simulink model "ACFT11_a_121_precoast_backup"  (R2026a)
settings: Solver=ode15s  StopTime=2200  FixedStep=0.01  MaxStep=0.05  MinStep=1e-4  AbsTol=1e-4
model workspace (MAT data in the model file):
  op11 : opcond.OperatingPoint (value not decoded)
  op_trim1 : opcond.OperatingReport (value not decoded)
  op_trim12 : opcond.OperatingReport (value not decoded)
  op_trim15 : opcond.OperatingReport (value not decoded)
  op_trim16 : opcond.OperatingReport (value not decoded)
  op_trim17 : opcond.OperatingReport (value not decoded)
  op_trim18 : opcond.OperatingReport (value not decoded)
  op_trim2 : opcond.OperatingReport (value not decoded)
  op_trim20 : opcond.OperatingReport (value not decoded)
  op_trim21 : opcond.OperatingReport (value not decoded)
  op_trim22 : opcond.OperatingReport (value not decoded)
  op_trim23 : opcond.OperatingReport (value not decoded)
  op_trim24 : opcond.OperatingReport (value not decoded)
  op_trim25 : opcond.OperatingReport (value not decoded)
  op_trim29 : opcond.OperatingReport (value not decoded)
  op_trim3 : opcond.OperatingReport (value not decoded)
  op_trim30 : opcond.OperatingReport (value not decoded)
  op_trim4 : opcond.OperatingReport (value not decoded)
  op_trim40 : opcond.OperatingReport (value not decoded)
  op_trim42 : opcond.OperatingReport (value not decoded)
  op_trim5 : opcond.OperatingReport (value not decoded)
  op_trim50 : opcond.OperatingReport (value not decoded)
  op_trim7 : opcond.OperatingReport (value not decoded)
  op_trim9 : opcond.OperatingReport (value not decoded)
values from neighbouring files (symbols this model uses):
  b = min(1, 2*(1-frac))    [export_kml.m]    (also in flight_hud.m = chaseBack; inertiatensor62.m = 9.05; setup_bfl_analysis.m = 9.05; setup_fcs_sim.m = 9.05)
  c = bar_colors{min(k,numel(bar_colors))}    [analyze_bfl.m]    (also in ecef_eom_fcn.m = w_eb_b(3); inertiatensor62.m = 15.55; optimize_indi_gains.m = 15.55; restore_normal_fcs.m = 15.55)
  CL_AlphaDot = 0    [inertiatensor62.m]    (also in setup_bfl_analysis.m; setup_fcs_sim.m; setup_takeoff_fcs.m)
  Cm_AlphaDot = 0    [inertiatensor62.m]    (also in setup_bfl_analysis.m; setup_fcs_sim.m; setup_takeoff_fcs.m)
  ecef_x0 = [ [0;0;0]; ECEF_v0; ECEF_q0; ECEF_w0 ]    [setup_ecef.m]    (also in setup_fcs_sim.m = build_ecef_x0(FCS_h_cmd, FCS_V_cmd, 2*pi/180))
  F = convhull(pts)    [Visualization_Takeoff2.m]    (also in attitude_ribbon.m = {[1 2 3],[1 4 2],[1 4 3],[4 5 1]})
  FCS_aerospike_thrust = 250000.0    (= 250000)    [fcs_params.m]
  FCS_alpha_max = 16.0    (= 16)    [fcs_params.m]
  FCS_bank_max = 35.0    (= 35)    [fcs_params.m]
  FCS_da_max = 20.0    (= 20)    [fcs_params.m]
  FCS_de_max = 25.0    (= 25)    [fcs_params.m]
  FCS_dr_max = 25.0    (= 25)    [fcs_params.m]
  FCS_dt = 0.01    [fcs_params.m]
  FCS_g = 9.80665    [fcs_params.m]
  FCS_Gmin_p = 0.02    [fcs_params.m]
  FCS_Gmin_q = 0.02    [fcs_params.m]
  FCS_Gmin_r = 0.01    [fcs_params.m]
  FCS_h_gnd = 2.24    [fcs_params.m]
  FCS_hdot_max = 30.0    (= 30)    [fcs_params.m]
  FCS_hdot_td = 0.3    [fcs_params.m]
  FCS_Kalpha = 3.0    (= 3)    [fcs_params.m]
  FCS_Kalpha_lim = 2.0    (= 2)    [fcs_params.m]
  FCS_Kbeta = 2.0    (= 2)    [fcs_params.m]
  FCS_Kflare = 1.0    (= 1)    [fcs_params.m]
  FCS_Kgamma = 1.5    [fcs_params.m]
  FCS_Kh = 0.10    (= 0.1)    [fcs_params.m]
  FCS_Knz = 20.0    (= 20)    [fcs_params.m]
  FCS_Kp = 6.0    (= 6)    [fcs_params.m]
  FCS_Kphi = 3.0    (= 3)    [fcs_params.m]
  FCS_Kq = 5.0    (= 5)    [fcs_params.m]
  FCS_Kr = 4.0    (= 4)    [fcs_params.m]
  FCS_Ktheta = 2.0    (= 2)    [fcs_params.m]
  FCS_link_timeout = 1.0    (= 1)    [fcs_params.m]
  FCS_MODE_AUTO = 0    [fcs_params.m]
  FCS_Nfilt = 20.0    (= 20)    [fcs_params.m]
  FCS_Nz_max = 3.0    (= 3)    [fcs_params.m]
  FCS_Nz_min = -1.0    (= -1)    [fcs_params.m]
  FCS_Nz_zoom_tgt = 2.0    (= 2)    [fcs_params.m]
  FCS_p_max = 40.0    (= 40)    [fcs_params.m]
  FCS_q_max = 15.0    (= 15)    [fcs_params.m]
  FCS_qbar_hi = 6000.0    (= 6000)    [fcs_params.m]
  FCS_qbar_lo = 1000.0    (= 1000)    [fcs_params.m]
  FCS_r_max = 15.0    (= 15)    [fcs_params.m]
  FCS_relight_M_hi = 2.0    (= 2)    [fcs_params.m]
  FCS_relight_M_lo = 0.35    [fcs_params.m]
  FCS_relight_qbar = 3000.0    (= 3000)    [fcs_params.m]
  FCS_stick_detent = 0.03    [fcs_params.m]
  FCS_stick_p_scale = 60.0    (= 60)    [fcs_params.m]
  FCS_stick_q_scale = 15.0    (= 15)    [fcs_params.m]
  FCS_tau_flare = 3.0    (= 3)    [fcs_params.m]
  FCS_TECS_Kep = 0.25    [fcs_params.m]
  FCS_TECS_Ktp = 0.30    (= 0.3)    [fcs_params.m]
  FCS_theta_climb = 12.0    (= 12)    [fcs_params.m]
  FCS_theta_max = 30.0    (= 30)    [fcs_params.m]
  FCS_theta_min = -20.0    (= -20)    [fcs_params.m]
  FCS_theta_trim = 0.0    (= 0)    [fcs_params.m]
  FCS_thr_max = 1.0    (= 1)    [fcs_params.m]
  FCS_thr_min = 0.0    (= 0)    [fcs_params.m]
  FCS_thr_trim = 0.50    (= 0.5)    [fcs_params.m]
  FCS_V_rotate = 94.0    (= 94)    [fcs_params.m]
  FCS_Vmin = 60.0    (= 60)    [fcs_params.m]
  FF_rates = [0.0,              2.5,              5.0,             73.0,             78.0,              0.5]    [fcs_params.m]
  GS_Gp_tab = Cl_da * (S*b/Ixx)    [setup_gschedule.m]
  GS_Gq_tab = Cm_de * (S*c/Iyy)    [setup_gschedule.m]
  GS_Gr_tab = Cn_dr * (S*b/Izz)    [setup_gschedule.m]
  MASS_fuel_total = MASS_full - MASS_empty - MASS_orbiter    (= 14700)    [fcs_params.m]
  q = q/norm(q)    [build_ecef_x0.m]    (also in ecef_eom_fcn.m = state(7:10); ecef_out_fcn.m = state(7:10); setup_ecef.m; test_ecef_eom.m = state(7:10))
  r = [0;diff(xc)]/0.1    [analyze_control_authority.m]    (also in ecef_eom_fcn.m = sqrt(r_e(1)^2+r_e(2)^2+r_e(3)^2); ecef_weight_body.m = sqrt(x^2 + y^2 + z^2); export_kml.m = min(1, 2*frac); test_ecef_eom.m = sqrt(r_e(1)^2+r_e(2)^2+r_e(3)^2))
  y_cg = 0    [inertiatensor62.m]    (also in setup_bfl_analysis.m; setup_fcs_sim.m; setup_takeoff_fcs.m)
  z_cg = 0.0    (= 0)    [inertiatensor62.m]    (also in setup_bfl_analysis.m; setup_fcs_sim.m; setup_takeoff_fcs.m)
undefined symbols (not defined in the file or in its folder): DiscIntNeverNeededParam, EqM, GS_alpha_cl, GS_alpha_cm, GS_alpha_cn, GS_mach_cl, GS_mach_cm, GS_mach_cn, MIL, Moderate
libraries: aerolibconvert2 x20, simulink x7, aerolibfltsims x3, aerolibwind2 x3, aerolibanim x1, aerolibatmos2 x1, shareddyn x1, aerolibobsolete x1, sl_discontinuities x1
(part 3 of 4)

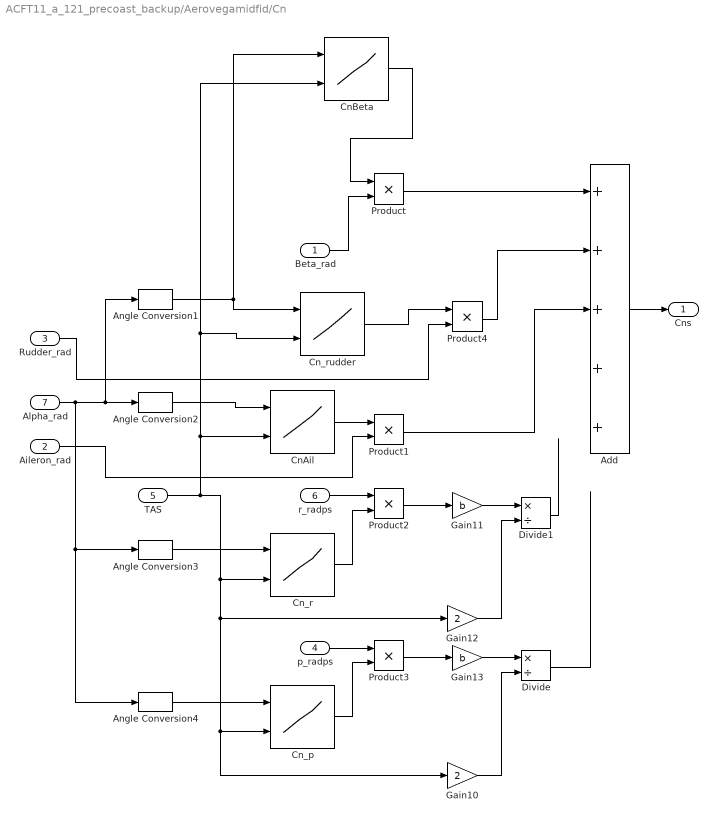
== system ACFT11_a_121_precoast_backup/Aerovegamidfid/Cn ==
  Beta_rad : Inport
  Aileron_rad : Inport  Port=2
  Rudder_rad : Inport  Port=3
  p_radps : Inport  Port=4
  TAS : Inport  Port=5
  r_radps : Inport  Port=6
  Alpha_rad : Inport  Port=7
  Add : Sum  Inputs=+++++
  Angle Conversion{1..4} (4 alike) : aerolibconvert2/Angle Conversion  IU=rad  OU=deg
  CnAil : Lookup_n-D  BreakpointsForDimension1=[-10;-5;0;5;10;15;20]  BreakpointsForDimension2=[0.40000000000000002;0.59999999999999998;0.80000000000000004;0.90000000000000002;0.94999999999999996;1;1.05;1.1000000000000001;1.1499999999999999;1.2;1.3999999999999999;1.6000000000000001;1.8;2;2.2000000000000002;2.3999999999999999;2.6000000000000001;2.7999999999999998;3;3.2000000000000002]  BreakpointsForDimension3=[10 20 30]  Table=[0.025618999999999999 0.032230000000000002 0.043424999999999998 0.047711000000000003 0.025152999999999998 0.0050109999999999998 0.001714 0.00056099999999999998 -0.00038000000000000002 -0.00101 -0.0044299999999999999 -0.0088500000000000002 -0.01047 -0.010330000000000001 -0.0096100000000000005 -0.0096100000000000005 -0.0082400000000000008 -0.0082400000000000008 -0.0071500000000000001 -0.0068300000000000001;0.032065999999999997 0.033909000000000002 0.043319999999999997 0.058770999999999997 0.036042999999999999 0.0046010000000000001 0.0010189999999999999 0.00039500000000000001 -0.00079000000000000001 -0.0035699999999999998 -0.0096299999999999997 -0.01081 -0.01025 -0.0091699999999999993 -0.0080800000000000004 -0.0072300000000000003 -0.0066100000000000004 -0.0060499999999999998 -0.0055199999999999997 -0.0049800000000000001;0.020569 0.023560999999999999 0.025321 0.020659 0.045733000000000003 0.0040819999999999997 -0.0057299999999999999 -0.0070600000000000003 -0.0085100000000000002 -0.0093799999999999994 -0.0097699999999999992 -0.0092499999999999995 -0.0081099999999999992 -0.00762 -0.0061399999999999996 -0.0053899999999999998 -0.00479 -0.0043099999999999996 -0.0039100000000000003 -0.0035100000000000001;0.014408000000000001 0.014364 0.0047060000000000001 0.032719999999999999 -0.0060200000000000002 -0.01091 -0.0031700000000000001 -0.0062700000000000004 -0.0082400000000000008 -0.0086899999999999998 -0.0077499999999999999 -0.0064700000000000001 -0.0057499999999999999 -0.0048300000000000001 -0.00413 -0.0035799999999999998 -0.00314 -0.0027899999999999999 -0.0025300000000000001 -0.0022300000000000002;-0.01451 0.0021649999999999998 0.011785 0.0099939999999999994 0.017096 0.012609 0.021628999999999999 0.01771 0.012371999999999999 0.0073509999999999999 0.00082600000000000002 -0.00048999999999999998 -0.00060999999999999997 -0.0010399999999999999 -0.0016100000000000001 -0.00158 -0.0015399999999999999 -0.0015900000000000001 -0.0016100000000000001 -0.0011100000000000001;-0.0029299999999999999 0.028791000000000001 0.014966999999999999 0.023009000000000002 0.023694 0.024584999999999999 0.021819000000000002 0.019778 0.017666999999999999 0.012969 0.0016080000000000001 0.00013999999999999999 6.6799999999999997e-05 7.8899999999999993e-05 -0.00042999999999999999 -0.00095 -0.00147 -0.0013500000000000001 -0.0015499999999999999 -0.00158;0.0069319999999999998 -0.0067799999999999996 0.001748 -0.0087899999999999992 0.019404999999999999 0.025475999999999999 0.020417000000000001 0.017842 0.015092 0.012945999999999999 0.0028990000000000001 0.00041800000000000002 -6.7000000000000002e-05 -0.00044999999999999999 -0.00088999999999999995 -0.00080999999999999996 -0.00101 -0.00109 -0.00117 -0.00080999999999999996]  InternalRulePriority=Speed  RndMeth=Simplest
      settings: InputPortMap=u0,u1
  CnBeta : Lookup_n-D  BreakpointsForDimension1=[-10;-5;0;5;10;15;20]  BreakpointsForDimension2=[0.40000000000000002;0.59999999999999998;0.80000000000000004;0.90000000000000002;0.94999999999999996;1;1.05;1.1000000000000001;1.1499999999999999;1.2;1.3999999999999999;1.6000000000000001;1.8;2;2.2000000000000002;2.3999999999999999;2.6000000000000001;2.7999999999999998;3;3.2000000000000002;3.3999999999999999;3.6000000000000001;3.7999999999999998;4]  Table=[0.047225000000000003 0.052442000000000003 0.072338 0.072338 0.072338 0.089275999999999994 0.095235 0.094727000000000006 0.092405000000000001 0.088535000000000003 0.078687999999999994 0.070837999999999998 0.061545999999999997 0.052052000000000001 0.046726999999999998 0.046726999999999998 0.04444 0.04444 0.037597999999999999 0.033663999999999999 0.033663999999999999 0.033663999999999999 0.033663999999999999 0.033663999999999999;0.055976999999999999 0.055794999999999997 0.053287000000000001 0.064735000000000001 0.081561999999999996 0.099891999999999995 0.095333000000000001 0.085306999999999994 0.075719999999999996 0.071434999999999998 0.085987999999999995 0.070606000000000002 0.056079999999999998 0.048198999999999999 0.046877000000000002 0.046877000000000002 0.040409 0.040409 0.032599999999999997 0.029361000000000002 0.025589000000000001 0.022336000000000002 0.01942 0.017468000000000001;0.042603000000000002 0.042603000000000002 0.048195000000000002 0.067723000000000005 0.073911000000000004 0.131243 0.089542999999999998 0.081192 0.075617000000000004 0.067141999999999993 0.056979000000000002 0.059299999999999999 0.051374999999999997 0.040273000000000003 0.031241999999999999 0.031241999999999999 0.021367000000000001 0.021367000000000001 0.016972000000000001 0.015805 0.013964000000000001 0.012834999999999999 0.012834999999999999 0.0090480000000000005;0.053624999999999999 0.057244999999999997 0.061199999999999997 0.064993999999999996 0.057278000000000003 0.12961600000000001 0.10612099999999999 0.10163 0.083560999999999996 0.072969999999999993 0.052317000000000002 0.045895999999999999 0.041921 0.034547000000000001 0.025399000000000001 0.025399000000000001 0.015058999999999999 0.015058999999999999 0.010803999999999999 0.0098340000000000007 0.0098340000000000007 0.008182 0.008182 0.0066670000000000002;-0.059130000000000002 -0.036020000000000003 0.055744000000000002 0.051433 0.049752999999999999 0.051705000000000001 0.055764000000000001 0.054408999999999999 0.058610000000000002 0.061033999999999998 0.056083000000000001 0.040585000000000003 0.046671999999999998 0.029899999999999999 0.026093000000000002 0.026093000000000002 0.018697999999999999 0.018697999999999999 0.015757 0.014958000000000001 0.013683000000000001 0.013683000000000001 0.013683000000000001 0.013683000000000001;0.073567999999999995 0.073567999999999995 0.049260999999999999 0.082597000000000004 0.063562999999999995 0.105932 0.10280599999999999 0.093148999999999996 0.086785000000000001 0.078143000000000004 0.066612000000000005 0.047106000000000002 0.037848 0.030197000000000002 0.024729999999999999 0.024729999999999999 0.020267 0.020267 0.019040000000000001 0.018467999999999998 0.018467999999999998 0.014066 0.012291 0.010137999999999999;0.043372000000000001 0.043372000000000001 -0.031040000000000002 0.062727000000000005 0.101004 0.074541999999999997 0.076042999999999999 0.076627000000000001 0.073422000000000001 0.068245 0.060051 0.056735000000000001 0.045987 0.034201000000000002 0.026283000000000001 0.026283000000000001 0.015492000000000001 0.015492000000000001 0.012355 0.012945 0.012945 0.011245 0.010423 0.010423]  InternalRulePriority=Speed  RndMeth=Simplest
      settings: InputPortMap=u0,u1
  Cn_p : Lookup_n-D  BreakpointsForDimension1=[-4;4;12;20]  BreakpointsForDimension2=[134;809]  Table=[0.1118776 0.0532406;-0.0280082 -0.0173089;-0.1713669 -0.0875218;-0.3112158 -0.1560315]  InternalRulePriority=Speed  RndMeth=Simplest
      settings: InputPortMap=u0,u1
  Cn_r : Lookup_n-D  BreakpointsForDimension1=[-4;4;12;20]  BreakpointsForDimension2=[134;809]  Table=[-0.1192202 -0.1053294;-0.118715 -0.0878488;-0.119394 -0.0686585;-0.1236918 -0.0481319]  InternalRulePriority=Speed  RndMeth=Simplest
      settings: InputPortMap=u0,u1
  Cn_rudder : Lookup_n-D  BreakpointsForDimension1=[-5;0;5;10;15;20]  BreakpointsForDimension2=[0.40000000000000002;0.59999999999999998;0.80000000000000004;0.90000000000000002;0.94999999999999996;1;1.05;1.1000000000000001;1.1499999999999999;1.2;1.3999999999999999;1.6000000000000001;1.8;2;2.2000000000000002;2.3999999999999999;2.6000000000000001;2.7999999999999998;3;3.2000000000000002;3.3999999999999999;3.6000000000000001;3.7999999999999998;4]  BreakpointsForDimension3=[10 20 30]  Table=[-0.061620000000000001 -0.063089999999999993 -0.062190000000000002 -0.062190000000000002 -0.062190000000000002 -0.057520000000000002 -0.05305 -0.049579999999999999 -0.046010000000000002 -0.042880000000000001 -0.03372 -0.028039999999999999 -0.024340000000000001 -0.021870000000000001 -0.019949999999999999 -0.018360000000000001 -0.017170000000000001 -0.016230000000000001 -0.015570000000000001 -0.015570000000000001 -0.014160000000000001 -0.01376 -0.013429999999999999 -0.013180000000000001;-0.057270000000000001 -0.058209999999999998 -0.059209999999999999 -0.053710000000000001 -0.053710000000000001 -0.052880000000000003 -0.054199999999999998 -0.051670000000000001 -0.048750000000000002 -0.045940000000000002 -0.035369999999999999 -0.028879999999999999 -0.024479999999999998 -0.021049999999999999 -0.018509999999999999 -0.016570000000000001 -0.014970000000000001 -0.01372 -0.012760000000000001 -0.012760000000000001 -0.01102 -0.01051 -0.01008 -0.0097800000000000005;-0.060850000000000001 -0.063789999999999999 -0.06232 -0.06232 -0.06232 -0.044010000000000001 -0.037379999999999997 -0.035709999999999999 -0.035709999999999999 -0.045240000000000002 -0.03483 -0.028240000000000001 -0.022839999999999999 -0.01908 -0.016199999999999999 -0.014069999999999999 -0.01257 -0.011429999999999999 -0.010489999999999999 -0.010489999999999999 -0.0088900000000000003 -0.0083499999999999998 -0.0079399999999999991 -0.0075900000000000004;-0.050169999999999999 -0.06003 -0.053019999999999998 -0.05459 -0.05459 -0.05459 -0.046460000000000001 -0.045019999999999998 -0.042040000000000001 -0.039390000000000001 -0.030200000000000001 -0.023810000000000001 -0.017950000000000001 -0.0146 -0.01247 -0.0115 -0.010670000000000001 -0.0097000000000000003 -0.0089599999999999992 -0.0089599999999999992 -0.00762 -0.0071199999999999996 -0.0067099999999999998 -0.0064200000000000004;-0.039649999999999998 -0.045130000000000003 -0.050880000000000002 -0.050880000000000002 -0.050880000000000002 -0.05348 -0.049509999999999998 -0.04582 -0.041689999999999998 -0.03678 -0.027119999999999998 -0.020809999999999999 -0.016539999999999999 -0.01355 -0.01133 -0.0094699999999999993 -0.0094699999999999993 -0.0094699999999999993 -0.0075700000000000003 -0.0075700000000000003 -0.0065700000000000003 -0.0061700000000000001 -0.0058199999999999997 -0.0055199999999999997;0 -0.036409999999999998 -0.049200000000000001 -0.044740000000000002 -0.060510000000000001 -0.055840000000000001 -0.049979999999999997 -0.046179999999999999 -0.042099999999999999 -0.036450000000000003 -0.024279999999999999 -0.018360000000000001 -0.014319999999999999 -0.0118 -0.0099399999999999992 -0.0086899999999999998 -0.0074700000000000001 -0.0074700000000000001 -0.0074700000000000001 -0.0074700000000000001 -0.0053099999999999996 -0.00513 -0.0048399999999999997 0]  InternalRulePriority=Speed  RndMeth=Simplest
      settings: InputPortMap=u0,u1
  Divide : Product  Inputs=*/
  Divide1 : Product  Inputs=*/
  Gain10 : Gain  Gain=2
  Gain11 : Gain  Gain=b
  Gain12 : Gain  Gain=2
  Gain13 : Gain  Gain=b
  Product{,1..4} (5 alike) : Product
  Cns : Outport
  wires:
  CnBeta/1 -> Product/1
  TAS/1 -> Cn_p/2, Gain10/1, Gain12/1, Cn_r/2, CnBeta/2, Cn_rudder/2, CnAil/2
  p_radps/1 -> Product3/1
  Angle Conversion1/1 -> CnBeta/1, Cn_rudder/1
  Aileron_rad/1 -> Product1/2
  Cn_p/1 -> Product3/2
  Angle Conversion3/1 -> Cn_r/1
  Alpha_rad/1 -> Angle Conversion4/1, Angle Conversion3/1, Angle Conversion2/1, Angle Conversion1/1
  CnAil/1 -> Product1/1
  Rudder_rad/1 -> Product4/2
  Angle Conversion2/1 -> CnAil/1
  Divide1/1 -> ?
  Angle Conversion4/1 -> Cn_p/1
  Add/1 -> Cns/1
  Cn_r/1 -> Product2/2
  Beta_rad/1 -> Product/2
  Cn_rudder/1 -> Product4/1
  Gain10/1 -> Divide/2
  Product4/1 -> Add/2
  r_radps/1 -> Product2/1
  Product2/1 -> Gain11/1
  Product/1 -> Add/1
  Product1/1 -> Add/3
  Product3/1 -> Gain13/1
  Gain11/1 -> Divide1/1
  Gain12/1 -> Divide1/2
  Gain13/1 -> Divide/1
  Divide/1 -> ?

== system ACFT11_a_121_precoast_backup/Aerovegamidfid/Cx ==
  Alpha_rad : Inport
  Elevator_rad : Inport  Port=2
  mach : Inport  Port=3
  Abs : Abs  SaturateOnIntegerOverflow=off
  Abs1 : Abs  SaturateOnIntegerOverflow=off
  Add : Sum
  Angle Conversion2 : aerolibconvert2/Angle Conversion  IU=rad  OU=deg
  Angle Conversion3 : aerolibconvert2/Angle Conversion  IU=rad  OU=deg
  CD : Scope
      settings: ActiveDisplayYMinimum=0.00115  ActiveDisplayYMaximum=0.06015  DataLoggingVariableName=ScopeData3
  Cx : Lookup_n-D  BreakpointsForDimension1=[-10;-5;0;5;10;15;20]  BreakpointsForDimension2=[0;0.40000000000000002;0.59999999999999998;0.80000000000000004;0.90000000000000002;0.94999999999999996;1;1.05;1.1000000000000001;1.1499999999999999;1.2;1.3999999999999999;1.6000000000000001;1.8;2;2.2000000000000002;2.3999999999999999;2.6000000000000001;2.7999999999999998;3;3.2000000000000002;3.3999999999999999;3.6000000000000001;3.7999999999999998;4]  Table=[0.015176 0.015176 0.011377999999999999 0.0057990000000000003 -0.0023999999999999998 -0.00911 -0.024819999999999998 -0.028649999999999998 -0.027179999999999999 -0.025260000000000001 -0.025020000000000001 -0.023939999999999999 -0.02384 -0.02299 -0.02164 -0.02043 -0.019550000000000001 -0.018700000000000001 -0.017989999999999999 -0.017510000000000001 -0.017639999999999999 -0.017639999999999999 -0.017639999999999999 -0.017639999999999999 -0.017639999999999999;-0.0017700000000000001 -0.0017700000000000001 -0.00214 -0.0030100000000000001 -0.0071599999999999997 -0.0161 -0.031660000000000001 -0.037170000000000002 -0.035540000000000002 -0.03286 -0.032030000000000003 -0.029790000000000001 -0.028400000000000002 -0.026620000000000001 -0.024580000000000001 -0.022790000000000001 -0.021489999999999999 -0.02026 -0.019210000000000001 -0.018440000000000002 -0.018270000000000002 -0.018409999999999999 -0.017770000000000001 -0.016750000000000001 -0.01669;-0.0088400000000000006 -0.0088400000000000006 -0.0092099999999999994 -0.0096500000000000006 -0.012319999999999999 -0.019640000000000001 -0.036339999999999997 -0.042209999999999998 -0.040779999999999997 -0.03814 -0.03705 -0.033430000000000001 -0.031109999999999999 -0.029100000000000001 -0.027019999999999999 -0.025049999999999999 -0.02341 -0.021839999999999998 -0.02052 -0.019529999999999999 -0.019179999999999999 -0.018780000000000002 -0.018780000000000002 -0.017260000000000001 -0.016650000000000002;-0.0014599999999999999 -0.0014599999999999999 -0.0024299999999999999 -0.0040099999999999997 -0.01414 -0.01856 -0.02877 -0.036159999999999998 -0.035220000000000001 -0.03338 -0.032280000000000003 -0.029100000000000001 -0.027140000000000001 -0.02588 -0.024510000000000001 -0.023210000000000001 -0.022179999999999998 -0.02104 -0.02001 -0.019230000000000001 -0.019050000000000001 -0.019220000000000001 -0.01857 -0.018020000000000001 -0.017520000000000001;0.012845000000000001 0.012845000000000001 0.011466 0.0064530000000000004 0.0020430000000000001 -0.00445 -0.020320000000000001 -0.026849999999999999 -0.026069999999999999 -0.02435 -0.024889999999999999 -0.024049999999999998 -0.023349999999999999 -0.02264 -0.022069999999999999 -0.021559999999999999 -0.021100000000000001 -0.020500000000000001 -0.019900000000000001 -0.019480000000000001 -0.01958 -0.019980000000000001 -0.019550000000000001 -0.019189999999999999 -0.018540000000000001;0.027647999999999999 0.027647999999999999 0.021609 0.012803999999999999 0.0070400000000000003 -0.0019599999999999999 -0.018159999999999999 -0.022790000000000001 -0.0229 -0.020920000000000001 -0.022100000000000002 -0.02281 -0.023140000000000001 -0.022780000000000002 -0.02222 -0.0218 -0.021530000000000001 -0.02111 -0.020760000000000001 -0.020590000000000001 -0.02094 -0.021690000000000001 -0.021690000000000001 -0.02129 -0.02112;0.039897000000000002 0.039897000000000002 0.028426 0.015706000000000001 0.0068849999999999996 -0.00562 -0.021430000000000001 -0.02291 -0.022769999999999999 -0.021219999999999999 -0.022589999999999999 -0.023449999999999999 -0.024420000000000001 -0.023699999999999999 -0.02316 -0.02282 -0.022550000000000001 -0.022280000000000001 -0.022079999999999999 -0.022079999999999999 -0.022759999999999999 -0.022759999999999999 -0.023810000000000001 -0.023789999999999999 -0.023800000000000002]  InternalRulePriority=Speed  RndMeth=Simplest
      settings: InputPortMap=u0,u1
  Cxelev : Lookup_n-D  BreakpointsForDimension1=[-10;-5;0;5;10;15;20]  BreakpointsForDimension2=[0;0.40000000000000002;0.59999999999999998;0.80000000000000004;0.90000000000000002;0.94999999999999996;1;1.05;1.1000000000000001;1.1499999999999999;1.2;1.3999999999999999;1.6000000000000001;1.8;2;2.2000000000000002;2.3999999999999999;2.6000000000000001;2.7999999999999998;3;3.2000000000000002;3.3999999999999999;3.6000000000000001;3.7999999999999998;4]  Table=[-0.0046499999999999996 -0.0046499999999999996 -0.0032699999999999999 -0.025829999999999999 -0.0040400000000000002 -0.017899999999999999 0.001769 0.011247999999999999 0.01295 0.015106 0.015151 0.013192000000000001 0.011768000000000001 0.012734000000000001 0.011769 0.010376 0.010376 0.0082279999999999992 0.0082279999999999992 0.0069090000000000002 0.0059410000000000001 0.0059410000000000001 0.0059410000000000001 0.0059410000000000001 0.0059410000000000001;-0.0066800000000000002 -0.0066800000000000002 -0.0060699999999999999 -0.025010000000000001 -0.027060000000000001 -0.017149999999999999 -0.0012899999999999999 0.0037989999999999999 0.0047809999999999997 0.0060959999999999999 0.0068279999999999999 0.006378 0.0060520000000000001 0.0065389999999999997 0.0058609999999999999 0.0048580000000000003 0.0041279999999999997 0.0036449999999999998 0.0033700000000000002 0.0031410000000000001 0.002944 0.002647 0.0025500000000000002 0.0024020000000000001 0.0022560000000000002;-0.00054000000000000001 -0.00054000000000000001 -0.0011100000000000001 -0.0043099999999999996 -0.0061999999999999998 -0.028840000000000001 -0.011259999999999999 -0.0018 -0.00027999999999999998 0.0013990000000000001 0.0025990000000000002 0.002078 0.0010839999999999999 0.001219 -0.0021099999999999999 0.00072599999999999997 0.00036699999999999998 0.00013100000000000001 -1.2e-05 -9.7999999999999997e-05 -0.00011 -8.5000000000000006e-05 -0.00020000000000000001 -8.7000000000000001e-05 -3.3000000000000003e-05;0.0022039999999999998 0.0022039999999999998 -0.00299 -0.01172 -0.040460000000000003 0.0010189999999999999 0.0023289999999999999 -0.0073899999999999999 -0.00547 -0.0043800000000000002 -0.0030899999999999999 -0.0022799999999999999 -0.0033600000000000001 -0.00364 -0.0035599999999999998 -0.00347 -0.0034099999999999998 -0.0033600000000000001 -0.00329 -0.0031800000000000001 -0.0030400000000000002 -0.0027100000000000002 -0.0026099999999999999 -0.0025400000000000002 -0.0023700000000000001;-0.0093799999999999994 -0.0093799999999999994 -0.0059300000000000004 -0.0166 -0.02145 -0.01976 -0.0089700000000000005 -0.016639999999999999 -0.01451 -0.013180000000000001 -0.01119 -0.0088500000000000002 -0.0083300000000000006 -0.0092099999999999994 -0.0089499999999999996 -0.0083199999999999993 -0.0076699999999999997 -0.0072199999999999999 -0.0065300000000000002 -0.00613 -0.0056299999999999996 -0.00528 -0.0050299999999999997 -0.0047200000000000002 -0.0045799999999999999;-0.013259999999999999 -0.013259999999999999 -0.017909999999999999 -0.027230000000000001 -0.02937 -0.028250000000000001 -0.023740000000000001 -0.023740000000000001 -0.0235 -0.022460000000000001 -0.020979999999999999 -0.01455 -0.012869999999999999 -0.01336 -0.012109999999999999 -0.01197 -0.010869999999999999 -0.01008 -0.0093699999999999999 -0.0087299999999999999 -0.0081899999999999994 -0.0078100000000000001 -0.0073800000000000003 -0.00745 -0.0070200000000000002;-0.01413 -0.01413 -0.021319999999999999 -0.0051399999999999996 -0.018419999999999999 -0.025250000000000002 -0.029909999999999999 -0.028039999999999999 -0.02579 -0.023230000000000001 -0.02257 -0.01823 -0.017309999999999999 -0.016469999999999999 -0.015440000000000001 -0.014789999999999999 -0.014500000000000001 -0.01362 -0.012699999999999999 -0.01201 -0.01171 -0.01091 -0.010619999999999999 -0.01038 -0.0097400000000000004]  InternalRulePriority=Speed  RndMeth=Simplest
      settings: InputPortMap=u0,u1
  Product1 : Product
  CDs : Outport
  wires:
  Angle Conversion3/1 -> Cxelev/1
  Angle Conversion2/1 -> Cx/1
  Add/1 -> CD/1, CDs/1
  Cxelev/1 -> Product1/1
  Abs1/1 -> Product1/2
  Elevator_rad/1 -> Abs1/1
  mach/1 -> Cxelev/2, Cx/2
  Abs/1 -> Angle Conversion3/1, Angle Conversion2/1
  Product1/1 -> Add/2
  Alpha_rad/1 -> Abs/1
  Cx/1 -> Add/1

== system ACFT11_a_121_precoast_backup/Aerovegamidfid/Cz ==
  Alpha_rad : Inport
  Elevator_rad : Inport  Port=2
  AlphaDot_radps : Inport  Port=3
  q_radps : Inport  Port=4
  mach : Inport  Port=5
  Add : Sum  Inputs=++++
  Angle Conversion : aerolibconvert2/Angle Conversion  IU=rad  OU=deg
  Angle Conversion1 : aerolibconvert2/Angle Conversion  IU=rad  OU=deg
  Angle Conversion2 : aerolibconvert2/Angle Conversion  IU=rad  OU=deg
  CL : Scope
      settings: ActiveDisplayYMinimum=-0.13493802926864251  ActiveDisplayYMaximum=0.70084486331652573  DataLoggingVariableName=ScopeData2
  CLq : Lookup_n-D  BreakpointsForDimension1=[-4;4;12;20]  BreakpointsForDimension2=[0.4;3.2]  Table=[1.2288323 0.5355072;1.2713015 0.5534266;1.332595 0.5496451;1.4098042 0.5244903]  InternalRulePriority=Speed  RndMeth=Simplest
      settings: InputPortMap=u0,u1
  Cz : Lookup_n-D  BreakpointsForDimension1=[-10;-5;0;5;10;15;20]  BreakpointsForDimension2=[0;0.40000000000000002;0.59999999999999998;0.80000000000000004;0.90000000000000002;0.94999999999999996;1;1.05;1.1000000000000001;1.1499999999999999;1.2;1.3999999999999999;1.6000000000000001;1.8;2;2.2000000000000002;2.3999999999999999;2.6000000000000001;2.7999999999999998;3;3.2000000000000002;3.3999999999999999;3.6000000000000001;3.7999999999999998;4]  Table=[0.30567499999999997 0.30567499999999997 0.33540799999999998 0.36827599999999999 0.389071 0.38653500000000002 0.42072900000000002 0.41339999999999999 0.40184999999999998 0.39316000000000001 0.38224599999999997 0.34154299999999999 0.30893999999999999 0.28386699999999998 0.26341999999999999 0.24568000000000001 0.23013600000000001 0.216224 0.20383299999999999 0.192827 0.18313599999999999 0.18313599999999999 0.18313599999999999 0.18313599999999999 0.18313599999999999;0.142681 0.142681 0.14651600000000001 0.155474 0.165686 0.17847199999999999 0.205539 0.20788300000000001 0.202959 0.19834499999999999 0.19364400000000001 0.172156 0.15248999999999999 0.137462 0.12623400000000001 0.117689 0.110626 0.104382 0.098658999999999997 0.093616000000000005 0.088925000000000004 0.084600999999999996 0.080792000000000003 0.076920000000000002 0.074323;-0.0015399999999999999 -0.0015399999999999999 -0.0030100000000000001 -0.0070499999999999998 -0.01342 0.0037069999999999998 0.028712000000000001 0.029978000000000001 0.030119 0.028112000000000002 0.026280999999999999 0.018055000000000002 0.010312999999999999 0.0045500000000000002 0.00040200000000000001 -0.0021900000000000001 -0.0037200000000000002 -0.0043800000000000002 -0.0045199999999999997 -0.0044299999999999999 -0.0043800000000000002 -0.00413 -0.00413 -0.00379 -0.00363;-0.15004999999999999 -0.15004999999999999 -0.15606 -0.16624 -0.18461 -0.18822 -0.14122000000000001 -0.14521999999999999 -0.13869999999999999 -0.13597000000000001 -0.13636999999999999 -0.13425000000000001 -0.13308 -0.12986 -0.12587000000000001 -0.12128 -0.1164 -0.11137 -0.10639 -0.10161000000000001 -0.096920000000000006 -0.092689999999999995 -0.088779999999999998 -0.085269999999999999 -0.082019999999999996;-0.28587000000000001 -0.28587000000000001 -0.31119000000000002 -0.34042 -0.36507000000000001 -0.37217 -0.33981 -0.33861000000000002 -0.33113999999999999 -0.32721 -0.31919999999999998 -0.30431999999999998 -0.29055999999999998 -0.27618999999999999 -0.26117000000000001 -0.24660000000000001 -0.23311000000000001 -0.22078999999999999 -0.20963000000000001 -0.19977 -0.19056000000000001 -0.18273 -0.17548 -0.16894999999999999 -0.16123000000000001;-0.44194 -0.44194 -0.50468000000000002 -0.54451000000000005 -0.57777000000000001 -0.59374000000000005 -0.58796000000000004 -0.56808000000000003 -0.55103999999999997 -0.54300999999999999 -0.52963000000000005 -0.48720999999999998 -0.45301000000000002 -0.42309999999999998 -0.39583000000000002 -0.37109999999999999 -0.34938000000000002 -0.32995000000000002 -0.31336999999999998 -0.29937000000000002 -0.2863 -0.27629999999999999 -0.27629999999999999 -0.25796999999999998 -0.25041999999999998;-0.66681000000000001 -0.66681000000000001 -0.72904000000000002 -0.79010999999999998 -0.83308000000000004 -0.83423000000000003 -0.83489999999999998 -0.80884999999999996 -0.78651000000000004 -0.76863000000000004 -0.74524000000000001 -0.67535999999999996 -0.61797999999999997 -0.57037000000000004 -0.53000000000000003 -0.49603999999999998 -0.4672 -0.44207000000000002 -0.42077999999999999 -0.40277000000000002 -0.38718000000000002 -0.38718000000000002 -0.36443999999999999 -0.35459000000000002 -0.34604000000000001]  InternalRulePriority=Speed  RndMeth=Simplest
      settings: InputPortMap=u0,u1
  Czelev : Lookup_n-D  BreakpointsForDimension1=[-10;-5;0;5;10;15;20]  BreakpointsForDimension2=[0;0.40000000000000002;0.59999999999999998;0.80000000000000004;0.90000000000000002;0.94999999999999996;1;1.05;1.1000000000000001;1.1499999999999999;1.2;1.3999999999999999;1.6000000000000001;1.8;2;2.2000000000000002;2.3999999999999999;2.6000000000000001;2.7999999999999998;3;3.2000000000000002;3.3999999999999999;3.6000000000000001;3.7999999999999998;4]  BreakpointsForDimension3=[0;10;20;30]  Table=[-0.39831 -0.39831 -0.44949 -0.49525999999999998 -0.42621999999999999 -0.42895 -0.28188000000000002 -0.24676000000000001 -0.22997000000000001 -0.2114 -0.19628000000000001 -0.14501 -0.11323999999999999 -0.093759999999999996 -0.079649999999999999 -0.069239999999999996 -0.069239999999999996 -0.055399999999999998 -0.055399999999999998 -0.045359999999999998 -0.038649999999999997 -0.038649999999999997 -0.038649999999999997 -0.038649999999999997 -0.038649999999999997;-0.38929000000000002 -0.38929000000000002 -0.41254999999999997 -0.46205000000000002 -0.52690999999999999 -0.48448000000000002 -0.26182 -0.24857000000000001 -0.23155000000000001 -0.21009 -0.19094 -0.14766000000000001 -0.11781 -0.096689999999999998 -0.082129999999999995 -0.071160000000000001 -0.06275 -0.055480000000000002 -0.04913 -0.043650000000000001 -0.038269999999999998 -0.032750000000000001 -0.02989 -0.027199999999999998 -0.025149999999999999;-0.40662999999999999 -0.40662999999999999 -0.43008999999999997 -0.45556000000000002 -0.44590999999999997 -0.45395000000000002 -0.21925 -0.23937 -0.22081999999999999 -0.19930999999999999 -0.17971999999999999 -0.13633000000000001 -0.1109 -0.09103 -0.078509999999999996 -0.065720000000000001 -0.057450000000000001 -0.050939999999999999 -0.045560000000000003 -0.040899999999999999 -0.036110000000000003 -0.031280000000000002 -0.028369999999999999 -0.025860000000000001 -0.023720000000000001;-0.42204999999999998 -0.42204999999999998 -0.43079000000000001 -0.41929 -0.44349 -0.33693000000000001 -0.20571999999999999 -0.24481 -0.22450000000000001 -0.1991 -0.1779 -0.12791 -0.10305 -0.08516 -0.071499999999999994 -0.061449999999999998 -0.053740000000000003 -0.047730000000000002 -0.04283 -0.03875 -0.03474 -0.030710000000000001 -0.028060000000000002 -0.026339999999999999 -0.02469;-0.34179999999999999 -0.34179999999999999 -0.42291000000000001 -0.46296999999999999 -0.42258000000000001 -0.35785 -0.24704999999999999 -0.23504 -0.22228999999999999 -0.19886999999999999 -0.18043999999999999 -0.11798 -0.090410000000000004 -0.074899999999999994 -0.063839999999999994 -0.055690000000000003 -0.049549999999999997 -0.044880000000000003 -0.041540000000000001 -0.039019999999999999 -0.037280000000000001 -0.033550000000000003 -0.032289999999999999 -0.031019999999999999 -0.029850000000000002;-0.33428999999999998 -0.33428999999999998 -0.48061999999999999 -0.46106999999999998 -0.48686000000000001 -0.33199000000000001 -0.25718999999999997 -0.23511000000000001 -0.21310999999999999 -0.19436999999999999 -0.17455999999999999 -0.11677999999999999 -0.083349999999999994 -0.070440000000000003 -0.062440000000000002 -0.059110000000000003 -0.05525 -0.051360000000000003 -0.048550000000000003 -0.046519999999999999 -0.043880000000000002 -0.04199 -0.040969999999999999 -0.039730000000000001 -0.039359999999999999;-0.38006000000000001 -0.38006000000000001 -0.39155000000000001 -0.51959999999999995 -0.56186000000000003 -0.26800000000000002 -0.24107000000000001 -0.22350999999999999 -0.21418999999999999 -0.20241999999999999 -0.18332999999999999 -0.13109000000000001 -0.097949999999999995 -0.077979999999999994 -0.069290000000000004 -0.065689999999999998 -0.064159999999999995 -0.061629999999999997 -0.059740000000000001 -0.057669999999999999 -0.056189999999999997 -0.053400000000000003 -0.052010000000000001 -0.05058 -0.04965]  InternalRulePriority=Speed  RndMeth=Simplest
      settings: InputPortMap=u0,u1
  Divide : Product  Inputs=*/
  Divide1 : Product  Inputs=*/
  Gain2 : Gain  Gain=CL_AlphaDot
  Gain4 : Gain  Gain=c
  Gain5 : Gain  Gain=2
  Gain6 : Gain  Gain=c
  Gain7 : Gain  Gain=2
  Product1 : Product
  Product2 : Product
  CLs : Outport
  wires:
  Divide/1 -> ?
  Divide1/1 -> Add/3
  Alpha_rad/1 -> Angle Conversion/1, Angle Conversion1/1, Angle Conversion2/1
  Angle Conversion2/1 -> CLq/1
  AlphaDot_radps/1 -> Gain2/1
  mach/1 -> Cz/2, CLq/2, Gain5/1, Gain7/1, Czelev/2
  Elevator_rad/1 -> Product1/2
  Angle Conversion/1 -> Cz/1
  Angle Conversion1/1 -> Czelev/1
  Gain7/1 -> Divide1/2
  Gain2/1 -> Gain6/1
  Czelev/1 -> Product1/1
  Gain6/1 -> Divide1/1
  q_radps/1 -> Product2/1
  CLq/1 -> Product2/2
  Product2/1 -> Gain4/1
  Product1/1 -> Add/2
  Add/1 -> CL/1, CLs/1
  Gain4/1 -> Divide/1
  Gain5/1 -> Divide/2
  Cz/1 -> Add/1

== system ACFT11_a_121_precoast_backup/Aerovegamidfid/L_25%2CG ==
  Y_Aero_N : Inport
  Z_Aero_N : Inport  Port=2
  Lb_Nm : Inport  Port=3
  Add : Sum  Inputs=--+
  Product7 : Product
  Product8 : Product
  y_CG_m : Constant  Value=y_cg
  z_CG_m : Constant  Value=z_cg
  L_Aero_Nm : Outport
  wires:
  Z_Aero_N/1 -> Product8/1
  Y_Aero_N/1 -> Product7/1
  y_CG_m/1 -> Product8/2
  Add/1 -> L_Aero_Nm/1  "L_Aero_Nm"
  Lb_Nm/1 -> Add/3
  Product7/1 -> Add/1
  Product8/1 -> Add/2
  z_CG_m/1 -> Product7/2

== system ACFT11_a_121_precoast_backup/Aerovegamidfid/M_25%2CG ==
  X_Aero_N : Inport
  Z_Aero_N : Inport  Port=2
  CG_mac : Inport  Port=3
  Mb_Nm : Inport  Port=4
  Add : Sum  Inputs=-++
  Fcn : Fcn  Expr=(u(1)-0.5287)*c
  Product5 : Product
  Product6 : Product
  z_CG_m : Constant  Value=z_cg
  M_Aero_Nm : Outport
  wires:
  z_CG_m/1 -> Product6/2
  Product6/1 -> Add/2
  Add/1 -> M_Aero_Nm/1  "M_Aero_Nm"
  X_Aero_N/1 -> Product6/1
  Z_Aero_N/1 -> Product5/1
  Product5/1 -> Add/1
  Fcn/1 -> Product5/2
  CG_mac/1 -> Fcn/1
  Mb_Nm/1 -> Add/3

== system ACFT11_a_121_precoast_backup/Aerovegamidfid/N_25%2CG ==
  X_Aero_N : Inport
  Y_Aero_N : Inport  Port=2
  CG_mac : Inport  Port=3
  Nb_Nm : Inport  Port=4
  Add : Sum  Inputs=-++
  Fcn1 : Fcn  Expr=(u(1)-0.5287)*c
  Product6 : Product
  Product7 : Product
  y_CG_m : Constant  Value=y_cg
  N_Aero_Nm : Outport
  wires:
  Product7/1 -> Add/2
  y_CG_m/1 -> Product7/2
  Add/1 -> N_Aero_Nm/1  "N_Aero_Nm"
  Nb_Nm/1 -> Add/3
  Fcn1/1 -> Product6/2
  Product6/1 -> Add/1
  X_Aero_N/1 -> Product7/1
  CG_mac/1 -> Fcn1/1
  Y_Aero_N/1 -> Product6/1

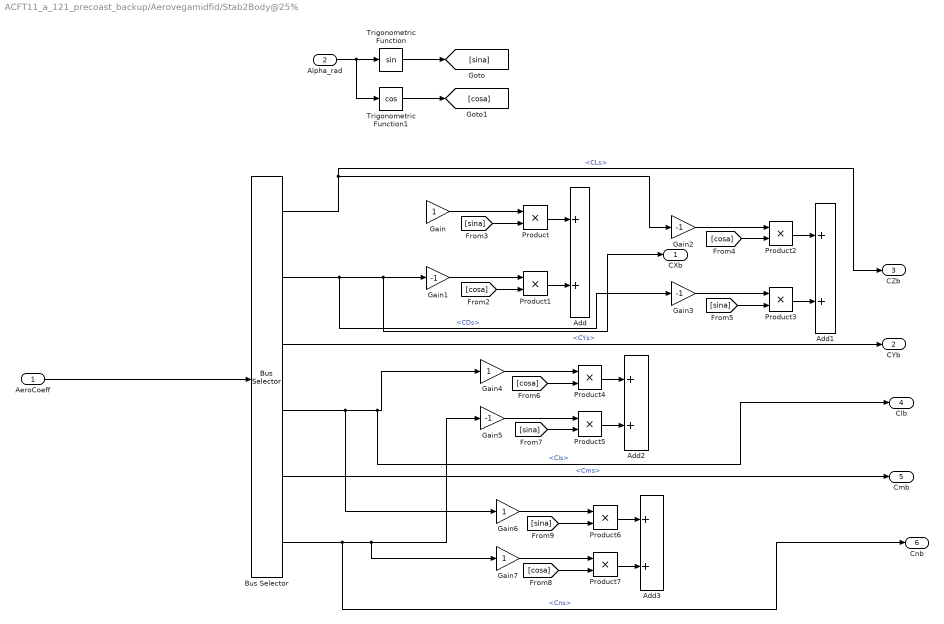
== system ACFT11_a_121_precoast_backup/Aerovegamidfid/Stab2Body@25% ==
  AeroCoeff : Inport
  Alpha_rad : Inport  Port=2
  Add{,1..3} (4 alike) : Sum
  Bus Selector : BusSelector  OutputSignals=CLs,CDs,CYs,Cls,Cms,Cns
  Gain{,4,6..7} (4 alike) : Gain
  Gain{1..3,5} (4 alike) : Gain  Gain=-1
  Product{,1..7} (8 alike) : Product
  Trigonometric Function : Trigonometry
  Trigonometric Function1 : Trigonometry  Operator=cos
  CXb : Outport
  CYb : Outport  Port=2
  CZb : Outport  Port=3
  Clb : Outport  Port=4
  Cmb : Outport  Port=5
  Cnb : Outport  Port=6
  wires:
  AeroCoeff/1 -> Bus Selector/1
  Alpha_rad/1 -> Trigonometric Function1/1, Trigonometric Function/1
  Trigonometric Function/1 -> [sina]
  Trigonometric Function1/1 -> [cosa]
  [sina] -> Product/2
  Bus Selector/1 -> CZb/1, Gain2/1  "<CLs>"
  Gain/1 -> Product/1
  [cosa] -> Product1/2
  Bus Selector/2 -> Gain3/1, CXb/1, Gain1/1  "<CDs>"
  Gain1/1 -> Product1/1
  Product1/1 -> Add/2
  Product/1 -> Add/1
  Gain2/1 -> Product2/1
  Gain3/1 -> Product3/1
  Product3/1 -> Add1/2
  Product2/1 -> Add1/1
  [sina] -> Product3/2
  [cosa] -> Product2/2
  Bus Selector/3 -> CYb/1  "<CYs>"
  Bus Selector/5 -> Cmb/1  "<Cms>"
  [cosa] -> Product4/2
  Gain4/1 -> Product4/1
  Gain5/1 -> Product5/1
  Product4/1 -> Add2/1
  Product5/1 -> Add2/2
  Bus Selector/4 -> Gain6/1, Clb/1, Gain4/1  "<Cls>"
  Bus Selector/6 -> Cnb/1, Gain7/1, Gain5/1  "<Cns>"
  [sina] -> Product5/2
  [sina] -> Product6/2
  Gain6/1 -> Product6/1
  Gain7/1 -> Product7/1
  Product6/1 -> Add3/1
  Product7/1 -> Add3/2
  [cosa] -> Product7/2

== system ACFT11_a_121_precoast_backup/Atmospheric/TAS2CAS ==
  Pressure_Pa : Inport
  Mach : Inport  Port=2
  (Gamma-1)/2 : Gain  Gain=(1.4-1)/2
  (Gamma-1)/Gamma : Constant  Value=(1.4-1)/1.4
  2*a0^2/(Gamma-1) : Gain  Gain=(2*340.262^2)/(1.4-1)
  Add2 : Sum
  Add3 : Sum  Inputs=+-
  Add4 : Sum
  Add5 : Sum  Inputs=+-
  Constant2 : Constant
  Divide5 : Product  Inputs=**
  Divide6 : Product  Inputs=*/
  Gamma/(Gamma-1) : Constant  Value=1.4/(1.4-1)
  Math Function2 : Math  Operator=square  SignedPower=on
  Math Function3 : Math  Operator=pow  SignedPower=on
  Math Function4 : Math  Operator=pow  SignedPower=on
  P0_Pa : Constant  Value=101325
  Sqrt2 : Sqrt
  CAS_mps : Outport
  wires:
  Sqrt2/1 -> CAS_mps/1
  2*a0^2/(Gamma-1)/1 -> Sqrt2/1
  Add5/1 -> 2*a0^2/(Gamma-1)/1
  Math Function4/1 -> Add5/1
  (Gamma-1)/Gamma/1 -> Math Function4/2
  Add4/1 -> Math Function4/1
  Divide6/1 -> Add4/1
  P0_Pa/1 -> Divide6/2
  Divide5/1 -> Divide6/1  "pt-ps"
  Pressure_Pa/1 -> Divide5/1
  Math Function3/1 -> Add3/1
  Add3/1 -> Divide5/2
  Gamma/(Gamma-1)/1 -> Math Function3/2
  Add2/1 -> Math Function3/1
  Constant2/1 -> Add5/2, Add4/2, Add3/2, Add2/2
  (Gamma-1)/2/1 -> Add2/1
  Mach/1 -> Math Function2/1
  Math Function2/1 -> (Gamma-1)/2/1

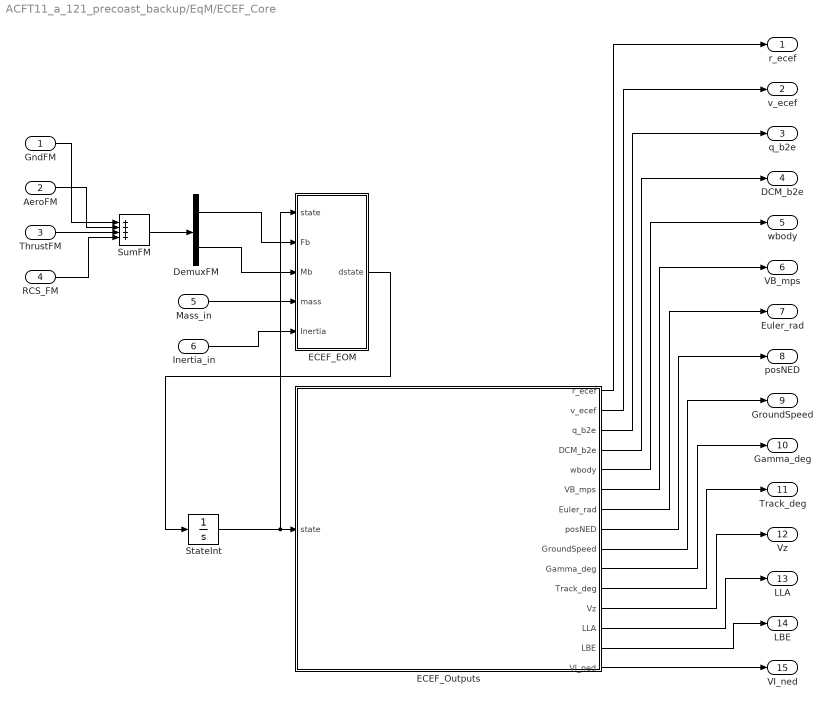
== system ACFT11_a_121_precoast_backup/EqM/ECEF_Core ==
  GndFM : Inport
  AeroFM : Inport  Port=2
  ThrustFM : Inport  Port=3
  RCS_FM : Inport  Port=4
  Mass_in : Inport  Port=5
  Inertia_in : Inport  Port=6
  DemuxFM : Demux  Outputs=[3 3]
  ECEF_EOM : MATLAB Function  TreatAsAtomicUnit=on
  ECEF_Outputs : MATLAB Function  TreatAsAtomicUnit=on
  StateInt : Integrator  InitialCondition=ecef_x0
  SumFM : Sum  Inputs=++++
  r_ecef : Outport
  v_ecef : Outport  Port=2
  q_b2e : Outport  Port=3
  DCM_b2e : Outport  Port=4
  wbody : Outport  Port=5
  VB_mps : Outport  Port=6
  Euler_rad : Outport  Port=7
  posNED : Outport  Port=8
  GroundSpeed : Outport  Port=9
  Gamma_deg : Outport  Port=10
  Track_deg : Outport  Port=11
  Vz : Outport  Port=12
  LLA : Outport  Port=13
  LBE : Outport  Port=14
  VI_ned : Outport  Port=15
  wires:
  Mass_in/1 -> ECEF_EOM/4(mass)
  ECEF_Outputs/12(Vz) -> Vz/1
  ThrustFM/1 -> SumFM/3
  ECEF_Outputs/8(posNED) -> posNED/1
  GndFM/1 -> SumFM/1
  DemuxFM/2 -> ECEF_EOM/3(Mb)
  RCS_FM/1 -> SumFM/4
  ECEF_Outputs/10(Gamma_deg) -> Gamma_deg/1
  AeroFM/1 -> SumFM/2
  SumFM/1 -> DemuxFM/1
  DemuxFM/1 -> ECEF_EOM/2(Fb)
  Inertia_in/1 -> ECEF_EOM/5(Inertia)
  StateInt/1 -> ECEF_Outputs/1(state), ECEF_EOM/1(state)
  ECEF_EOM/1(dstate) -> StateInt/1
  ECEF_Outputs/1(r_ecef) -> r_ecef/1
  ECEF_Outputs/2(v_ecef) -> v_ecef/1
  ECEF_Outputs/3(q_b2e) -> q_b2e/1
  ECEF_Outputs/4(DCM_b2e) -> DCM_b2e/1
  ECEF_Outputs/5(wbody) -> wbody/1
  ECEF_Outputs/6(VB_mps) -> VB_mps/1
  ECEF_Outputs/7(Euler_rad) -> Euler_rad/1
  ECEF_Outputs/9(GroundSpeed) -> GroundSpeed/1
  ECEF_Outputs/11(Track_deg) -> Track_deg/1
  ECEF_Outputs/13(LLA) -> LLA/1
  ECEF_Outputs/14(LBE) -> LBE/1
  ECEF_Outputs/15(VI_ned) -> VI_ned/1

== system ACFT11_a_121_precoast_backup/EqM/ExtForcesMoments ==
  Mass_kg : Inport
  GroundForcesMoments_N_Nm : Inport  Port=2
  AeroForcesMoments_N_Nm : Inport  Port=3
  ThrustForcesMoments_N_Nm : Inport  Port=4
  RCS_forces and moments : Inport  Port=5
  r_ecef_m : Inport  Port=6
  DCM_b2e : Inport  Port=7
  Add : Sum  Inputs=++++
  Demux : Demux  Outputs=2
  Demux1 : Demux  Outputs=3
  Divide : Product  Inputs=*/  Multiplication=Matrix(*)
  Gain : Gain  Gain=-1
  GravityBody : MATLAB Function  TreatAsAtomicUnit=on
  Mux1 : Mux  Inputs=3
  Scope{,1..4} (5 alike) : Scope
      Scope settings: ActiveDisplayYMinimum=-1  ActiveDisplayYMaximum=1  DataLoggingVariableName=ScopeData3
      Scope1 settings: ActiveDisplayYMinimum=-82844.26507  ActiveDisplayYMaximum=35036.98226  DataLoggingVariableName=ScopeData4
      Scope2 settings: ActiveDisplayYMinimum=-76487.985446301493  ActiveDisplayYMaximum=104454.47273578765  DataLoggingVariableName=ScopeData51
      Scope3 settings: ActiveDisplayYMinimum=-1  ActiveDisplayYMaximum=1  DataLoggingVariableName=ScopeData52
      Scope4 settings: ActiveDisplayYMinimum=-1  ActiveDisplayYMaximum=1  DataLoggingVariableName=ScopeData53
  Sum : Sum  Inputs=|++
  ExtForces_N : Outport
  ExtMoments_Nm : Outport  Port=2
  LoadFactors : Outport  Port=3
  wires:
  Sum/1 -> ExtForces_N/1
  Divide/1 -> Demux1/1
  ThrustForcesMoments_N_Nm/1 -> Add/3, Scope3/1
  Add/1 -> Scope/1, Demux/1
  Demux1/1 -> Mux1/1  "nx"
  Demux1/2 -> Mux1/2  "ny"
  AeroForcesMoments_N_Nm/1 -> Add/2, Scope2/1
  Mux1/1 -> LoadFactors/1
  Demux1/3 -> Gain/1
  Gain/1 -> Mux1/3  "nz"
  Demux/2 -> ExtMoments_Nm/1  "Moments"
  GroundForcesMoments_N_Nm/1 -> Scope1/1, Add/1
  Demux/1 -> Divide/1, Sum/2  "Forces"
  RCS_forces and moments/1 -> Scope4/1, Add/4
  r_ecef_m/1 -> GravityBody/1(r_ecef)
  DCM_b2e/1 -> GravityBody/2(DCM_b2e)
  Mass_kg/1 -> GravityBody/3(mass)
  GravityBody/1(Fw_body) -> Sum/1
  GravityBody/2(W_mag) -> Divide/2

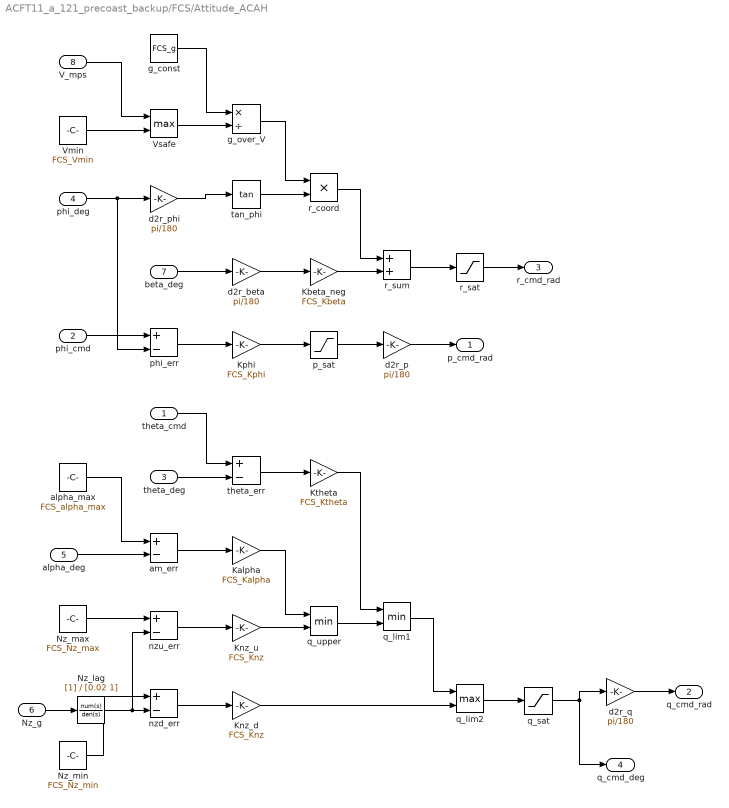
== system ACFT11_a_121_precoast_backup/FCS/Attitude_ACAH ==
  theta_cmd : Inport
  phi_cmd : Inport  Port=2
  theta_deg : Inport  Port=3
  phi_deg : Inport  Port=4
  alpha_deg : Inport  Port=5
  Nz_g : Inport  Port=6
  beta_deg : Inport  Port=7
  V_mps : Inport  Port=8
  Kalpha : Gain  Gain=FCS_Kalpha
  Kbeta_neg : Gain  Gain=FCS_Kbeta
  Knz_d : Gain  Gain=FCS_Knz
  Knz_u : Gain  Gain=FCS_Knz
  Kphi : Gain  Gain=FCS_Kphi
  Ktheta : Gain  Gain=FCS_Ktheta
  Nz_lag : TransferFcn  Denominator=[0.02 1]
  Nz_max : Constant  Value=FCS_Nz_max
  Nz_min : Constant  Value=FCS_Nz_min
  Vmin : Constant  Value=FCS_Vmin
  Vsafe : MinMax  Function=max  Inputs=2
  alpha_max : Constant  Value=FCS_alpha_max
  am_err : Sum  Inputs=+-
  d2r_beta : Gain  Gain=pi/180
  d2r_p : Gain  Gain=pi/180
  d2r_phi : Gain  Gain=pi/180
  d2r_q : Gain  Gain=pi/180
  g_const : Constant  Value=FCS_g
  g_over_V : Product  Inputs=*/
  nzd_err : Sum  Inputs=+-
  nzu_err : Sum  Inputs=+-
  p_sat : Saturate  UpperLimit=FCS_p_max  LowerLimit=-FCS_p_max
  phi_err : Sum  Inputs=+-
  q_lim1 : MinMax  Inputs=2
  q_lim2 : MinMax  Function=max  Inputs=2
  q_sat : Saturate  UpperLimit=FCS_q_max  LowerLimit=-FCS_q_max
  q_upper : MinMax  Inputs=2
  r_coord : Product  Inputs=**
  r_sat : Saturate  UpperLimit=FCS_r_max*pi/180  LowerLimit=-FCS_r_max*pi/180
  r_sum : Sum
  tan_phi : Trigonometry  Operator=tan
  theta_err : Sum  Inputs=+-
  p_cmd_rad : Outport
  q_cmd_rad : Outport  Port=2
  r_cmd_rad : Outport  Port=3
  q_cmd_deg : Outport  Port=4
  wires:
  r_sat/1 -> r_cmd_rad/1
  r_sum/1 -> r_sat/1
  Kbeta_neg/1 -> r_sum/2
  r_coord/1 -> r_sum/1
  d2r_beta/1 -> Kbeta_neg/1
  beta_deg/1 -> d2r_beta/1
  tan_phi/1 -> r_coord/2
  g_over_V/1 -> r_coord/1
  Vsafe/1 -> g_over_V/2
  g_const/1 -> g_over_V/1
  Vmin/1 -> Vsafe/2
  V_mps/1 -> Vsafe/1
  d2r_phi/1 -> tan_phi/1
  d2r_p/1 -> p_cmd_rad/1
  p_sat/1 -> d2r_p/1
  Kphi/1 -> p_sat/1
  phi_err/1 -> Kphi/1
  phi_deg/1 -> phi_err/2, d2r_phi/1
  phi_cmd/1 -> phi_err/1
  d2r_q/1 -> q_cmd_rad/1
  q_sat/1 -> q_cmd_deg/1, d2r_q/1
  q_lim2/1 -> q_sat/1
  Knz_d/1 -> q_lim2/2
  q_lim1/1 -> q_lim2/1
  q_upper/1 -> q_lim1/2
  Ktheta/1 -> q_lim1/1
  Knz_u/1 -> q_upper/2
  Kalpha/1 -> q_upper/1
  nzd_err/1 -> Knz_d/1
  Nz_min/1 -> nzd_err/1
  nzu_err/1 -> Knz_u/1
  Nz_max/1 -> nzu_err/1
  am_err/1 -> Kalpha/1
  alpha_deg/1 -> am_err/2
  alpha_max/1 -> am_err/1
  theta_err/1 -> Ktheta/1
  theta_deg/1 -> theta_err/2
  theta_cmd/1 -> theta_err/1
  Nz_g/1 -> Nz_lag/1
  Nz_lag/1 -> nzu_err/2, nzd_err/2

== system ACFT11_a_121_precoast_backup/FCS/HeadingHold ==
  track : Inport
  psi_cmd : Inport  Port=2
  V : Inport  Port=3
  qbar : Inport  Port=4
  L1law : MATLAB Function  TreatAsAtomicUnit=on
  bank_sat : Saturate  UpperLimit=FCS_bank_max  LowerLimit=-FCS_bank_max
  phi_cmd : Outport
  wires:
  L1law/1(phi) -> bank_sat/1
  V/1 -> L1law/3(V)
  track/1 -> L1law/2(track)
  psi_cmd/1 -> L1law/1(psi_cmd)
  bank_sat/1 -> phi_cmd/1
  qbar/1 -> L1law/4(qbar)
